simulink model "pid_ctrl"  (R2024a)
settings: Solver=FixedStepDiscrete  StartTime=0.0  StopTime=10  FixedStep=0.02  RelTol=1e-3
settings Model: Creator=bai  LastModifiedBy=bai
settings OptimizationCC: DefaultParameterBehavior=Inlined  EnhancedBackFolding=on  PassReuseOutputArgsAs=Individual arguments  ZeroExternalMemoryAtStartup=off  ZeroInternalMemoryAtStartup=off  OptimizeBlockOrder=speed  DifferentSizesBufferReuse=on  OptimizationCustomize=off  EfficientTunableParamExpr=on
settings DebuggingCC: ParameterTunabilityLossMsg=error
settings SFSimCC: MATLABDynamicMemAlloc=off
settings RTWCC: Description=Embedded Coder  SystemTargetFile=ert.tlc  GenCodeOnly=on  TemplateMakefile=ert_default_tmf  GenerateReport=on  TargetLang=C++
settings CodeAppCC: ForceParamTrailComments=on  IgnoreCustomStorageClasses=off  OperatorAnnotations=on  SimulinkDataObjDesc=on  SFDataObjDesc=on  InsertBlockDesc=on
settings ERTTargetCC: TargetLangStandard=C++11 (ISO)  CodeInterfacePackaging=C++ class  InlinedParameterPlacement=NonHierarchical  RootIOFormat=Structure reference  ERTCustomFileTemplate=example_file_process.tlc

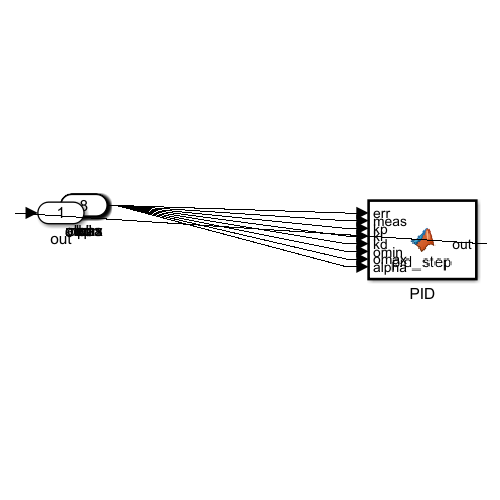
[thumbnail: Simulink's stored preview of the top-level diagram]
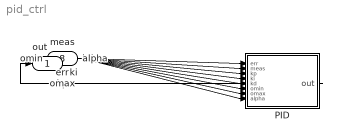
== system pid_ctrl ==
  err : Inport
  meas : Inport  Port=2
  kp : Inport  Port=3
  ki : Inport  Port=4
  kd : Inport  Port=5
  omin : Inport  Port=6
  omax : Inport  Port=7
  alpha : Inport  Port=8
  PID : MATLAB Function  TreatAsAtomicUnit=on
  out : Outport
  wires:
  err/1 -> PID/1(err)
  meas/1 -> PID/2(meas)
  kp/1 -> PID/3(kp)
  ki/1 -> PID/4(ki)
  kd/1 -> PID/5(kd)
  omin/1 -> PID/6(omin)
  omax/1 -> PID/7(omax)
  alpha/1 -> PID/8(alpha)
  PID/1(out) -> out/1

== matlab function pid_ctrl/PID ==
  data: err input; out output; meas input; kp input; ki input; kd input; omin input; omax input; alpha input
function out = pid_step(err, meas, kp, ki, kd, omin, omax, alpha)
% 与 C++ Pid::update 同一算法，dt 固定为 0.02
dt = 0.02;
persistent integ prev dfilt first
if isempty(integ), integ = 0; prev = 0; dfilt = 0; first = true; end

dterm = 0;
if ~first
    raw = -(meas - prev) / dt;
    dfilt = dfilt + alpha * (raw - dfilt);
    dterm = kd * dfilt;
end
prev = meas;  first = false;

p = kp * err;
cand = integ + err * dt;
unsat = p + ki * cand + dterm;
out = min(max(unsat, omin), omax);

satHigh = unsat > omax && err > 0;
satLow  = unsat < omin && err < 0;
if ~(satHigh || satLow)
    integ = cand;
end
end
